simulink model "experiment_supervisor"  (R2026b)
settings: Solver=FixedStepDiscrete  StopTime=inf  FixedStep=Ts
model workspace (MAT data in the model file):
  CAN_ANGLE_DEG2ICUB = Simulink.Parameter
  CAN_ANGLE_DEG2ICUB.Value = 182.044449
  CAN_ANGLE_DEG2ICUB.Complexity = 'real'
  CAN_ANGLE_DEG2ICUB.Dimensions = [1 1]
  CAN_ANGLE_DEG2ICUB.DataType = 'single'
  CAN_ANGLE_ICUB2DEG = Simulink.Parameter
  CAN_ANGLE_ICUB2DEG.Value = 0.00549316406
  CAN_ANGLE_ICUB2DEG.Complexity = 'real'
  CAN_ANGLE_ICUB2DEG.Dimensions = [1 1]
  CAN_ANGLE_ICUB2DEG.DataType = 'single'
  Ts = Simulink.Parameter
  Ts.Value = 0.01
  Ts.Complexity = 'real'
  Ts.Dimensions = [1 1]
  Ts.DocUnits = 's'
  board_ID = Simulink.Parameter
  board_ID.Value = 1
  board_ID.Complexity = 'real'
  board_ID.Dimensions = [1 1]
undefined symbols (not defined in the file or in its folder): canChannel
libraries: canmsglib x20, canlib x4, simulink x1
settings Model: DataDictionary=amcmj1.sldd  Creator=upattacini  LastModifiedBy=ksangalli
settings SolverCC: DecoupledContinuousIntegration=on  MinimalZcImpactIntegration=on
settings OptimizationCC: ReuseModelBlockBuffer=off  SimCompilerOptimization=on
settings DebuggingCC: ArithmeticOperatorsInVariantConditions=warning  ParameterPrecisionLossMsg=none
settings HardwareCC: ProdHWDeviceType=Intel->x86-64 (Linux 64)  ProdLongLongMode=on
settings SFSimCC: CustomCodeUndefinedFunction=UseInterfaceOnly  SimUseLocalCustomCode=off
settings RTWCC: DLArmComputeVersion=19.05  Description=Simulink Desktop Real-Time  RTWCompilerOptimization=on  RTWUseLocalCustomCode=off  SystemTargetFile=sldrt.tlc  TemplateMakefile=sldrt.tmf
settings SimulinkDesktopRealTimeCC: ParMdlRefBuildCompliant=on  RealTimeExecution=kernel  TargetLibSuffix=_sldrt.a  TargetPreCompLibLocation=C:\Program Files\MATLAB\R2026b\toolbox\sldrt\lib\win64

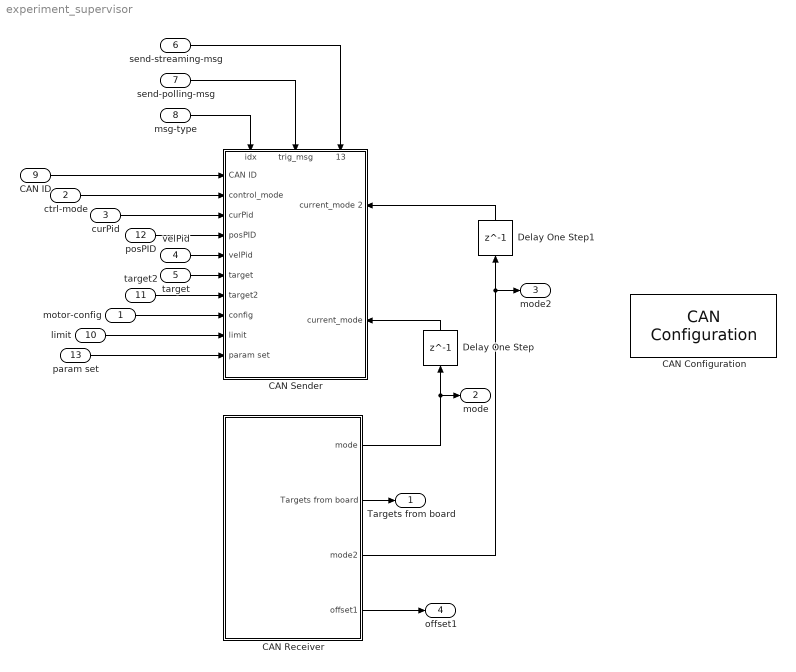
== system experiment_supervisor ==
  motor-config : Inport  OutDataTypeStr=Bus: MotorConfigurationExternal
  ctrl-mode : Inport  Port=2  OutDataTypeStr=Enum: MCControlModes
  curPid : Inport  Port=3  OutDataTypeStr=Bus: PID
  velPid : Inport  Port=4  OutDataTypeStr=Bus: PID
  target : Inport  Port=5
  send-streaming-msg : Inport  Port=6  OutDataTypeStr=uint8
  send-polling-msg : Inport  Port=7  OutDataTypeStr=uint8
  msg-type : Inport  Port=8  OutDataTypeStr=uint8
  CAN ID : Inport  Port=9
  limit : Inport  Port=10
  target2 : Inport  Port=11
  posPID : Inport  Port=12  OutDataTypeStr=Bus: PID
  param set : Inport  Port=13  OutDataTypeStr=Bus: MotorConfigurationExtSet
  CAN Configuration : canlib/CAN Configuration  BlockHandle=2987.0028  Device=Vector VN1610 1 (Channel 1)  DeviceMenu=Vector VN1610 1 (Channel 1)  ObjConstructor=canChannel('Vector', 'VN1610 1', 1)  BusSpeed=1000000  EnableBitParameters=off  SJW=1  TSEG1=4  TSEG2=3  NSamples=1  AckMode=Normal
  CAN Receiver : Subsystem
  CAN Sender : Subsystem
      settings: PortSchema="{\"entries\":[{\"content\":{\"sides\":[{\"content\":{\"connectorIds\":[\"In1\",\"In2\",\"In3\",\"In4\",\"In5\",\"In6\",\"In7\",\"In8\",\"In9\",\"In10\"]},\"type\":\"ConnectorPlacement.EquallySpacedRectSide\",\"uuid\":\"bdd6ce9e-9b65-4aba-9b48-f09f8c1326bb\"},{\"content\":{\"connectorIds\":[\"In14\",\"In15\"],\"side\":\"RIGHT\"},\"type\":\"ConnectorPlacement.EquallySpacedRectSide\",\"uuid\":\"141c9ef5-f742-47fc-b635-015c7474b58f\"},{\"content\":{\"connectorIds\":[\"In11\",\"In12\",\"In13\"],\"side\":\"TOP\"},\"type\":\"ConnectorPlacement.EquallySpacedRectSide\",\"uuid\":\"624889ac-74c5-4b05-9d21-0587daea952f\"}]},\"type\":\"ConnectorPlacement.EquallySpacedConnector\",\"uuid\":\"a748afda-e52d-41b4-a312-ee668058905d\"}],\"packageUris\":[\"http://schema.mathworks.com/mf0/Connector/R2020b\"],\"version\":\"1.0\"}"
  Delay One Step : Delay  DelayLength=1
  Delay One Step1 : Delay  DelayLength=1
  Targets from board : Outport
  mode : Outport  Port=2
  mode2 : Outport  Port=3
  offset1 : Outport  Port=4
  wires:
  ctrl-mode/1 -> CAN Sender/2(control_mode)
  send-streaming-msg/1 -> CAN Sender/13(trig_periodic)
  CAN Receiver/2(Targets from board) -> Targets from board/1
  velPid/1 -> CAN Sender/5(velPid)
  curPid/1 -> CAN Sender/3(curPid)
  motor-config/1 -> CAN Sender/8(config)
  CAN Receiver/1(mode) -> mode/1, Delay One Step/1
  Delay One Step/1 -> CAN Sender/15(current_mode)
  send-polling-msg/1 -> CAN Sender/12(trig_msg)
  msg-type/1 -> CAN Sender/11(idx)
  target/1 -> CAN Sender/6(target)
  CAN ID/1 -> CAN Sender/1(CAN ID)
  limit/1 -> CAN Sender/9(limit)
  CAN Receiver/4(offset1) -> offset1/1
  CAN Receiver/3(mode2) -> mode2/1, Delay One Step1/1
  Delay One Step1/1 -> CAN Sender/14(current_mode 2)
  target2/1 -> CAN Sender/7(target2)
  posPID/1 -> CAN Sender/4(posPID)
  param set/1 -> CAN Sender/10(param set)

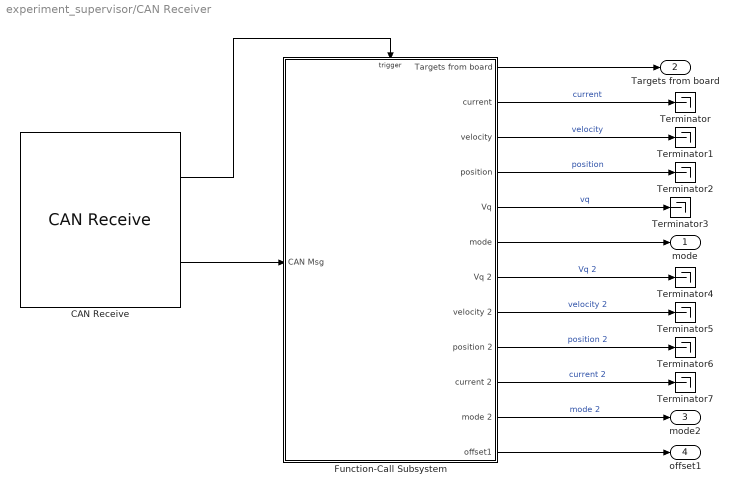
== system experiment_supervisor/CAN Receiver ==
  CAN Receive : canlib/CAN Receive  BlockHandle=2993.0018  Device=Vector VN1610 1 (Channel 1)  DeviceMenu=Vector VN1610 1 (Channel 1)  ObjConstructor=canChannel('Vector', 'VN1610 1', 1)  EnableStandardIDsFilter=off  StdIDsCombo=Allow all  StandardIDs=0  EnableExtendedIDsFilter=off  ExtIDsCombo=Allow all  ExtendedIDs=0  SampleTime=Ts  MsgsPerTimestep=all  InternalFilterUpdateStatus=on  BusOutput=on
  Function-Call Subsystem : Subsystem  TreatAsAtomicUnit=on
  Terminator{,1..7} (8 alike) : Terminator
  mode : Outport
  Targets from board : Outport  Port=2
  mode2 : Outport  Port=3
  offset1 : Outport  Port=4
  wires:
  CAN Receive/1 -> Function-Call Subsystem/Trigger
  CAN Receive/2 -> Function-Call Subsystem/1(CAN Msg)
  Function-Call Subsystem/2(current) -> Terminator/1  "current"
  Function-Call Subsystem/3(velocity) -> Terminator1/1  "velocity"
  Function-Call Subsystem/4(position) -> Terminator2/1  "position"
  Function-Call Subsystem/5(Vq) -> Terminator3/1  "vq"
  Function-Call Subsystem/1(Targets from board) -> Targets from board/1
  Function-Call Subsystem/6(mode) -> mode/1
  Function-Call Subsystem/7(Vq 2) -> Terminator4/1  "Vq 2"
  Function-Call Subsystem/8(velocity 2) -> Terminator5/1  "velocity 2"
  Function-Call Subsystem/9(position 2) -> Terminator6/1  "position 2"
  Function-Call Subsystem/10(current 2) -> Terminator7/1  "current 2"
  Function-Call Subsystem/11(mode 2) -> mode2/1  "mode 2"
  Function-Call Subsystem/12(offset1) -> offset1/1

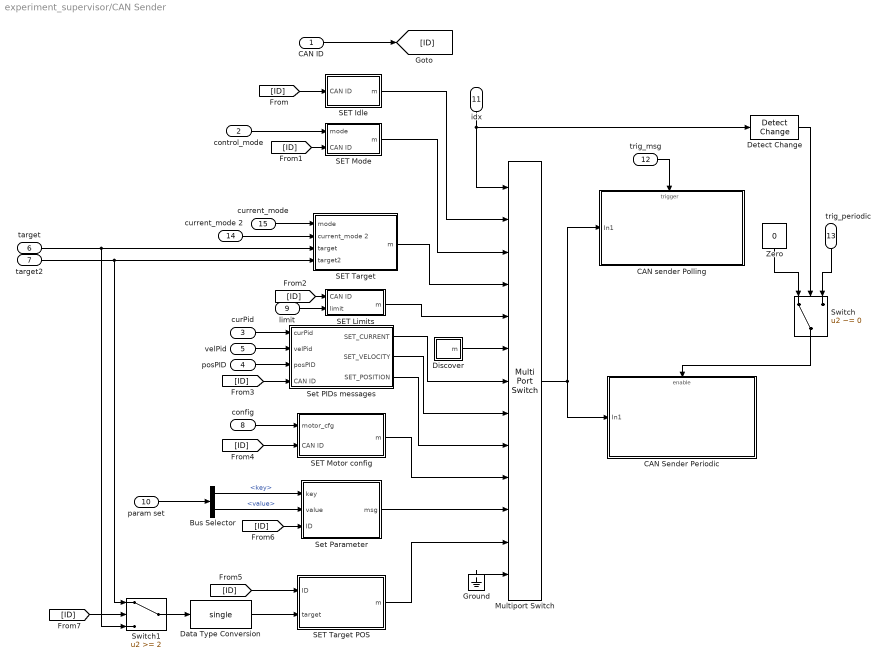
== system experiment_supervisor/CAN Sender ==
  CAN ID : Inport
  control_mode : Inport  Port=2
  curPid : Inport  Port=3
  posPID : Inport  Port=4
  velPid : Inport  Port=5
  target : Inport  Port=6
  target2 : Inport  Port=7
  config : Inport  Port=8
  limit : Inport  Port=9
  param set : Inport  Port=10  OutDataTypeStr=Bus: MotorConfigurationExtSet
  idx : Inport  Port=11
  trig_msg : Inport  Port=12
  trig_periodic : Inport  Port=13
  current_mode 2 : Inport  Port=14
  current_mode : Inport  Port=15
  Bus Selector : BusSelector  OutputSignals=key,value
  CAN Sender Periodic : Subsystem  TreatAsAtomicUnit=on
  CAN sender Polling : Subsystem
  Data Type Conversion : DataTypeConversion  OutDataTypeStr=single  SaturateOnIntegerOverflow=off  RndMeth=Floor
  Detect Change : simulink/Logic and Bit Operations/Detect Change  vinit=0  OutDataTypeStr=boolean
  Discover : Subsystem
  Ground : Ground
  Multiport Switch : MultiPortSwitch  Inputs=12  DiagnosticForDefault=Warning  SaturateOnIntegerOverflow=off  InputSameDT=off
  SET Idle : Subsystem
  SET Limits : Subsystem
  SET Mode : Subsystem
  SET Motor config : Subsystem
  SET Target : Subsystem
  "SET Target POS " : Subsystem
  Set PIDs messages : Subsystem
  Set Parameter : Subsystem
  Switch : Switch  Criteria=u2 ~= 0  SaturateOnIntegerOverflow=off  InputSameDT=off
  Switch1 : Switch  Threshold=2  SaturateOnIntegerOverflow=off  InputSameDT=off
  Zero : Constant  Value=0  OutDataTypeStr=Inherit: Inherit via back propagation
  wires:
  idx/1 -> Multiport Switch/1, Detect Change/1
  trig_msg/1 -> CAN sender Polling/Trigger
  trig_periodic/1 -> Switch/3
  Multiport Switch/1 -> CAN sender Polling/1(In1), CAN Sender Periodic/1(In1)
  Set PIDs messages/2(SET_VELOCITY) -> Multiport Switch/8
  Set PIDs messages/1(SET_CURRENT) -> Multiport Switch/7
  velPid/1 -> Set PIDs messages/2(velPid)
  curPid/1 -> Set PIDs messages/1(curPid)
  Detect Change/1 -> Switch/2
  Zero/1 -> Switch/1
  Switch/1 -> CAN Sender Periodic/Enable
  SET Limits/1(m) -> Multiport Switch/5
  current_mode/1 -> SET Target/1(mode)
  target/1 -> Switch1/3, SET Target/3(target)
  SET Target/1(m) -> Multiport Switch/4
  config/1 -> SET Motor config/1(motor_cfg)
  control_mode/1 -> SET Mode/1(mode)
  SET Mode/1(m) -> Multiport Switch/3
  SET Idle/1(m) -> Multiport Switch/2
  Discover/1(m) -> Multiport Switch/6
  [ID] -> SET Idle/1(CAN ID)
  [ID] -> SET Mode/2(CAN ID)
  [ID] -> SET Limits/1(CAN ID)
  [ID] -> Set PIDs messages/4(CAN ID)
  [ID] -> SET Motor config/2(CAN ID)
  CAN ID/1 -> [ID]
  limit/1 -> SET Limits/2(limit)
  current_mode 2/1 -> SET Target/2(current_mode 2)
  target2/1 -> Switch1/1, SET Target/4(target2)
  posPID/1 -> Set PIDs messages/3(posPID)
  [ID] -> "SET Target POS "/1(ID)
  "SET Target POS "/1(m) -> Multiport Switch/12
  Data Type Conversion/1 -> "SET Target POS "/2(target)
  Set PIDs messages/3(SET_POSITION) -> Multiport Switch/9
  SET Motor config/1(m) -> Multiport Switch/10
  param set/1 -> Bus Selector/1
  Ground/1 -> Multiport Switch/13
  Bus Selector/1 -> Set Parameter/1(key)  "<key>"
  Bus Selector/2 -> Set Parameter/2(value)  "<value>"
  [ID] -> Set Parameter/3(ID)
  Set Parameter/1(msg) -> Multiport Switch/11
  Switch1/1 -> Data Type Conversion/1
  [ID] -> Switch1/2

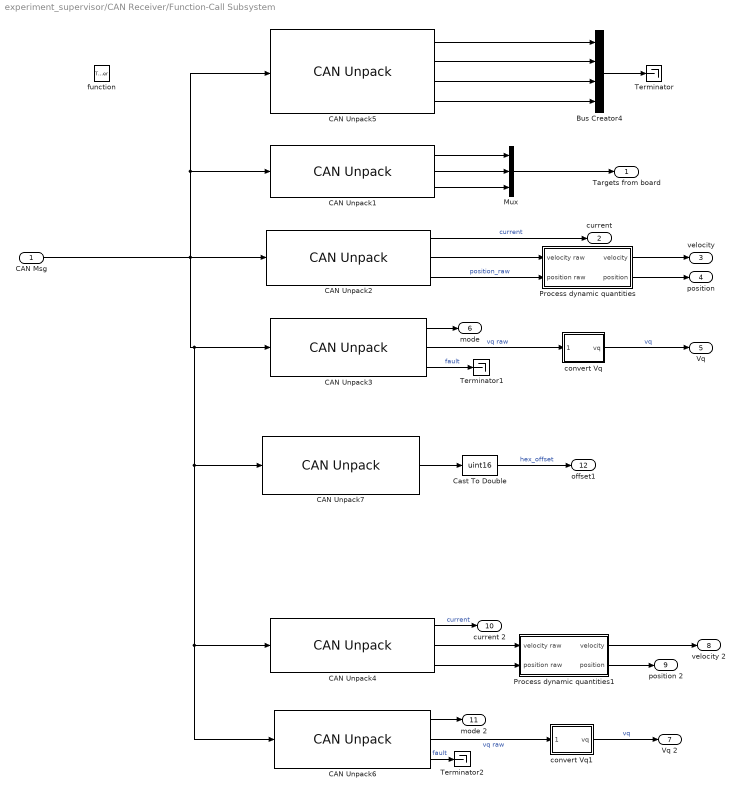
== system experiment_supervisor/CAN Receiver/Function-Call Subsystem ==
  CAN Msg : Inport
  function : TriggerPort  TriggerType=function-call  VariantControl=(inherit)
  Bus Creator4 : BusCreator  Inputs=4
  CAN Unpack1 : canmsglib/CAN Unpack  MsgList=(none)  MsgName=TARGETS  MsgIDType=Standard (11-bit identifier)  MsgIdentifier=0x10F  MsgLength=8  SignalInfo={ 'Target1', '0', '16', 'LE', 'signed', 'Standard', '0', '1', '0', '-Inf', 'Inf'; 'Target2', '16', '16', 'LE', 'signed', 'Standard', '0', '1', '0', '-Inf', 'Inf'; 'Target3', '32', '16', 'LE', 'signed', 'Standard', '0', '1', '0', '-Inf', 'Inf' }  IDPort=off  TimestampPort=off  ErrorPort=off  RemotePort=off  LengthPort=off  StatusPort=off  ApplyMinMax=off
  CAN Unpack2 : canmsglib/CAN Unpack  MsgList=(none)  MsgName=FOC  MsgIDType=Standard (11-bit identifier)  MsgIdentifier=0x110  MsgLength=8  SignalInfo={ 'current', '0', '16', 'LE', 'signed', 'Standard', '0', '1', '0', '-Inf', 'Inf'; 'velocity', '16', '16', 'LE', 'signed', 'Standard', '0', '1', '0', '-Inf', 'Inf'; 'position', '32', '32', 'LE', 'signed', 'Standard', '0', '1', '0', '-Inf', 'Inf' }  IDPort=off  TimestampPort=off  ErrorPort=off  RemotePort=off  LengthPort=off  StatusPort=off  ApplyMinMax=off
  CAN Unpack3 : canmsglib/CAN Unpack  MsgList=(none)  MsgName=STATUS  MsgIDType=Standard (11-bit identifier)  MsgIdentifier=0x113  MsgLength=8  SignalInfo={ 'mode', '0', '8', 'LE', 'unsigned', 'Standard', '0', '1', '0', '-Inf', 'Inf'; 'pwm', '16', '16', 'LE', 'unsigned', 'Standard', '0', '1', '0', '-Inf', 'Inf'; 'fault', '32', '8', 'LE', 'unsigned', 'Standard', '0', '1', '0', '-Inf', 'Inf' }  IDPort=off  TimestampPort=off  ErrorPort=off  RemotePort=off  LengthPort=off  StatusPort=off  ApplyMinMax=off
  CAN Unpack4 : canmsglib/CAN Unpack  MsgList=(none)  MsgName=FOC  MsgIDType=Standard (11-bit identifier)  MsgIdentifier=0x120  MsgLength=8  SignalInfo={ 'current', '0', '16', 'LE', 'signed', 'Standard', '0', '1', '0', '-Inf', 'Inf'; 'velocity', '16', '16', 'LE', 'signed', 'Standard', '0', '1', '0', '-Inf', 'Inf'; 'position', '32', '32', 'LE', 'signed', 'Standard', '0', '1', '0', '-Inf', 'Inf' }  IDPort=off  TimestampPort=off  ErrorPort=off  RemotePort=off  LengthPort=off  StatusPort=off  ApplyMinMax=off
  CAN Unpack5 : canmsglib/CAN Unpack  MsgList=(none)  MsgName=DISCOVER  MsgIDType=Standard (11-bit identifier)  MsgIdentifier=0x710  MsgLength=5  SignalInfo={}  IDPort=on  TimestampPort=on  ErrorPort=off  RemotePort=off  LengthPort=on  StatusPort=off  ApplyMinMax=off
      settings: DataFormat=raw data
  CAN Unpack6 : canmsglib/CAN Unpack  MsgList=(none)  MsgName=STATUS  MsgIDType=Standard (11-bit identifier)  MsgIdentifier=0x123  MsgLength=8  SignalInfo={ 'mode', '0', '8', 'LE', 'unsigned', 'Standard', '0', '1', '0', '-Inf', 'Inf'; 'pwm', '16', '16', 'LE', 'unsigned', 'Standard', '0', '1', '0', '-Inf', 'Inf'; 'fault', '32', '8', 'LE', 'unsigned', 'Standard', '0', '1', '0', '-Inf', 'Inf' }  IDPort=off  TimestampPort=off  ErrorPort=off  RemotePort=off  LengthPort=off  StatusPort=off  ApplyMinMax=off
  CAN Unpack7 : canmsglib/CAN Unpack  MsgList=(none)  MsgName=Debug  MsgIDType=Standard (11-bit identifier)  MsgIdentifier=0x119  MsgLength=8  SignalInfo={ 'offset', '0', '16', 'LE', 'unsigned', 'Standard', '0', '1', '0', '-Inf', 'Inf' }  IDPort=off  TimestampPort=off  ErrorPort=off  RemotePort=off  LengthPort=off  StatusPort=off  ApplyMinMax=off
  Cast To Double : DataTypeConversion  OutDataTypeStr=uint16  SaturateOnIntegerOverflow=off  RndMeth=Floor
  Mux : Mux  Inputs=3
  Process dynamic quantities : Subsystem
  Process dynamic quantities1 : Subsystem
  Terminator : Terminator
  Terminator1 : Terminator
  Terminator2 : Terminator
  convert Vq : Subsystem
  convert Vq1 : Subsystem
  Targets from board : Outport
  current : Outport  Port=2  Unit=mA
  velocity : Outport  Port=3  Unit=deg/s
  position : Outport  Port=4  Unit=deg
  Vq : Outport  Port=5  Unit=%  PortDimensions=1
  mode : Outport  Port=6  OutDataTypeStr=uint8
  Vq 2 : Outport  Port=7
  velocity 2 : Outport  Port=8
  position 2 : Outport  Port=9
  current 2 : Outport  Port=10  Unit=mA
  mode 2 : Outport  Port=11  OutDataTypeStr=uint8
  offset1 : Outport  Port=12
  wires:
  CAN Unpack5/4 -> Bus Creator4/4
  CAN Unpack5/3 -> Bus Creator4/3
  CAN Unpack5/2 -> Bus Creator4/2
  CAN Unpack5/1 -> Bus Creator4/1
  Bus Creator4/1 -> Terminator/1
  CAN Unpack1/1 -> Mux/1
  CAN Unpack1/2 -> Mux/2
  CAN Unpack1/3 -> Mux/3
  Mux/1 -> Targets from board/1
  CAN Unpack2/2 -> Process dynamic quantities/1(velocity raw)
  Process dynamic quantities/2(position) -> position/1
  Process dynamic quantities/1(velocity) -> velocity/1
  CAN Unpack2/3 -> Process dynamic quantities/2(position raw)  "position_raw"
  CAN Unpack3/2 -> convert Vq/1(vq raw)  "vq raw"
  CAN Unpack3/1 -> mode/1
  convert Vq/1(vq) -> Vq/1  "vq"
  CAN Unpack3/3 -> Terminator1/1  "fault"
  CAN Msg/1 -> CAN Unpack5/1, CAN Unpack1/1, CAN Unpack7/1, CAN Unpack6/1, CAN Unpack4/1, CAN Unpack3/1, CAN Unpack2/1
  CAN Unpack4/2 -> Process dynamic quantities1/1(velocity raw)
  CAN Unpack4/3 -> Process dynamic quantities1/2(position raw)
  CAN Unpack6/2 -> convert Vq1/1(vq raw)  "vq raw"
  Process dynamic quantities1/1(velocity) -> velocity 2/1
  Process dynamic quantities1/2(position) -> position 2/1
  convert Vq1/1(vq) -> Vq 2/1  "vq"
  CAN Unpack4/1 -> current 2/1  "current"
  CAN Unpack6/1 -> mode 2/1
  CAN Unpack6/3 -> Terminator2/1  "fault"
  CAN Unpack7/1 -> Cast To Double/1
  Cast To Double/1 -> offset1/1  "hex_offset"
  CAN Unpack2/1 -> current/1  "current"

== system experiment_supervisor/CAN Sender/CAN Sender Periodic ==
  In1 : Inport
  Enable : EnablePort
  CAN Transmit : canlib/CAN Transmit  BlockHandle=1809.0078  Device=Vector VN1610 1 (Channel 1)  DeviceMenu=Vector VN1610 1 (Channel 1)  ObjConstructor=canChannel('Vector', 'VN1610 1', 1)  EnableEventTransmit=off  EnablePeriodicTransmit=on  MessagePeriod=Ts
  wires:
  In1/1 -> CAN Transmit/1

== system experiment_supervisor/CAN Sender/CAN sender Polling ==
  In1 : Inport
  Trigger : TriggerPort  VariantControl=(inherit)  PortDimensions=1
  CAN Transmit : canlib/CAN Transmit  BlockHandle=1818.0078  Device=Vector VN1610 1 (Channel 1)  DeviceMenu=Vector VN1610 1 (Channel 1)  ObjConstructor=canChannel('Vector', 'VN1610 1', 1)  EnableEventTransmit=off  EnablePeriodicTransmit=off  MessagePeriod=1.000
  wires:
  In1/1 -> CAN Transmit/1

== system experiment_supervisor/CAN Sender/Discover ==
  CAN Pack4 : canmsglib/CAN Pack  MsgList=(none)  MsgName=DISCOVER  MsgIDType=Standard (11-bit identifier)  MsgIdentifier=0x70F  CANIDInput=off  MsgLength=1  Remote=off  ApplyMinMax=off  BusOutput=on  SignalInfo={}
      settings: DataFormat=raw data
  discover : Constant  Value=0xFF
  m : Outport
  wires:
  CAN Pack4/1 -> m/1
  discover/1 -> CAN Pack4/1

== system experiment_supervisor/CAN Sender/SET Idle ==
  CAN ID : Inport
  CAN Pack : canmsglib/CAN Pack  MsgList=(none)  MsgName=CAN Idle  MsgIDType=Standard (11-bit identifier)  MsgIdentifier=board_ID  CANIDInput=on  MsgLength=2  Remote=off  ApplyMinMax=off  BusOutput=on  SignalInfo={ 'Idle', '0', '16', 'LE', 'unsigned', 'Standard', '0', '1', '0', '-Inf', 'Inf' }
      settings: DataFormat=manually specified signals
  idle-mode : Constant  Value=0x09  OutDataTypeStr=Inherit: Inherit via back propagation
  m : Outport
  wires:
  idle-mode/1 -> CAN Pack/1
  CAN ID/1 -> CAN Pack/2
  CAN Pack/1 -> m/1

== system experiment_supervisor/CAN Sender/SET Limits ==
  CAN ID : Inport
  limit : Inport  Port=2
  CAN Pack3 : canmsglib/CAN Pack  MsgList=(none)  MsgName=CAN Limits  MsgIDType=Standard (11-bit identifier)  MsgIdentifier=board_ID  CANIDInput=on  MsgLength=8  Remote=off  ApplyMinMax=off  BusOutput=on  SignalInfo={ 'CMD', '0', '8', 'LE', 'unsigned', 'Standard', '0', '1', '0', '-Inf', 'Inf'; 'X', '8', '8', 'LE', 'unsigned', 'Standard', '0', '1', '0', '-Inf', 'Inf'; 'NOMINAL', '16', '16', 'LE', 'unsigned', 'Standard', '0', '1', '0', '-Inf', 'Inf'; 'PEAK', '32', '16', 'LE', 'unsigned', 'Standard', '0', '1', '0', '-Inf', 'Inf'; 'OVERLOAD', '48', '16', 'LE', 'unsigned', 'Standard', '0', '1', '0', '-Inf', 'Inf' }
      settings: DataFormat=manually specified signals
  Constant1 : Constant  Value=0x48  OutDataTypeStr=Inherit: Inherit via back propagation
  Constant2 : Constant  Value=0  OutDataTypeStr=Inherit: Inherit via back propagation
  Demux : Demux  Outputs=3
  m : Outport
  wires:
  Constant2/1 -> CAN Pack3/2
  Constant1/1 -> CAN Pack3/1
  Demux/1 -> CAN Pack3/3
  Demux/3 -> CAN Pack3/5
  Demux/2 -> CAN Pack3/4
  CAN ID/1 -> CAN Pack3/6
  CAN Pack3/1 -> m/1
  limit/1 -> Demux/1

== system experiment_supervisor/CAN Sender/SET Mode ==
  mode : Inport
  CAN ID : Inport  Port=2
  CAN Pack1 : canmsglib/CAN Pack  MsgList=(none)  MsgName=SET Control Mode  MsgIDType=Standard (11-bit identifier)  MsgIdentifier=board_ID  CANIDInput=on  MsgLength=2  Remote=off  ApplyMinMax=off  BusOutput=on  SignalInfo={ 'CMD', '0', '8', 'LE', 'unsigned', 'Standard', '0', '1', '0', '-Inf', 'Inf'; 'CTRL', '8', '8', 'LE', 'signed', 'Standard', '0', '1', '0', '-Inf', 'Inf' }
      settings: DataFormat=manually specified signals
  Cast : DataTypeConversion  OutDataTypeStr=uint8  SaturateOnIntegerOverflow=off  RndMeth=Floor
  current-mode : Constant  Value=0x09  OutDataTypeStr=Inherit: Inherit via back propagation
  m : Outport
  wires:
  current-mode/1 -> CAN Pack1/1
  Cast/1 -> CAN Pack1/2
  mode/1 -> Cast/1
  CAN ID/1 -> CAN Pack1/3
  CAN Pack1/1 -> m/1

== system experiment_supervisor/CAN Sender/SET Motor config ==
  motor_cfg : Inport
  CAN ID : Inport  Port=2
  CAN Pack5 : canmsglib/CAN Pack  MsgList=(none)  MsgName=Set_Motor_Config  MsgIDType=Standard (11-bit identifier)  MsgIdentifier=board_ID  CANIDInput=on  MsgLength=8  Remote=off  ApplyMinMax=off  BusOutput=on  SignalInfo={ 'CMD', '0', '8', 'LE', 'unsigned', 'Standard', '0', '1', '0', '-Inf', 'Inf'; 'FLAGS', '8', '8', 'LE', 'unsigned', 'Standard', '0', '1', '0', '-Inf', 'Inf'; 'RES_ENCODER', '16', '16', 'LE', 'signed', 'Standard', '0', '1', '0', '-Inf', 'Inf'; 'OFFSET_ENCODER', '32', '16', 'LE', 'signed', 'Standard', '0', '1', '0', '-Inf', 'Inf'; 'N_POLES', '48', '8', 'LE', 'unsigned', 'Standard', '0', '1', '0', '-Inf', 'Inf'; 'ENCODER_TOLERANCE', '56', '8', 'LE', 'unsigned', 'Standard', '0', '1', '0', '-Inf', 'Inf' }
      settings: DataFormat=manually specified signals
  Constant3 : Constant  Value=0x77  OutDataTypeStr=Inherit: Inherit via back propagation
  Unpack motor configuration : MATLAB Function  TreatAsAtomicUnit=on
  m : Outport
  wires:
  motor_cfg/1 -> Unpack motor configuration/1(motor_cfg)
  Unpack motor configuration/2(resolution) -> CAN Pack5/3
  Unpack motor configuration/3(rotor_offset) -> CAN Pack5/4
  Unpack motor configuration/1(flags) -> CAN Pack5/2
  Unpack motor configuration/4(n_poles) -> CAN Pack5/5
  Unpack motor configuration/5(enc_tolerance) -> CAN Pack5/6
  Constant3/1 -> CAN Pack5/1
  CAN ID/1 -> CAN Pack5/7
  CAN Pack5/1 -> m/1

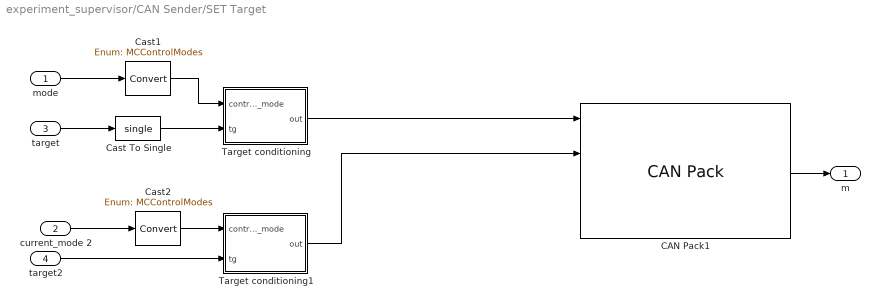
== system experiment_supervisor/CAN Sender/SET Target ==
  mode : Inport
  current_mode 2 : Inport  Port=2
  target : Inport  Port=3
  target2 : Inport  Port=4
  CAN Pack1 : canmsglib/CAN Pack  MsgList=(none)  MsgName=CAN Target  MsgIDType=Standard (11-bit identifier)  MsgIdentifier=0x10F  CANIDInput=off  MsgLength=8  Remote=off  ApplyMinMax=off  BusOutput=on  SignalInfo={ 'Target 1', '0', '16', 'LE', 'signed', 'Standard', '0', '1', '0', '-Inf', 'Inf'; 'Target 2', '16', '16', 'LE', 'signed', 'Standard', '0', '1', '0', '-Inf', 'Inf'; 'Target 3', '32', '16', 'LE', 'signed', 'Standard', '0', '1', '0', '-Inf', 'Inf'; 'Target 4', '48', '16', 'LE', 'signed', 'Standard', '0', '1', '0', '-Inf', 'Inf' }
      settings: DataFormat=manually specified signals
  Cast To Single : DataTypeConversion  OutDataTypeStr=single  SaturateOnIntegerOverflow=off  RndMeth=Floor
  Cast1 : DataTypeConversion  OutDataTypeStr=Enum: MCControlModes  SaturateOnIntegerOverflow=off  RndMeth=Floor
  Cast2 : DataTypeConversion  OutDataTypeStr=Enum: MCControlModes  SaturateOnIntegerOverflow=off  RndMeth=Floor
  Target conditioning : Subsystem
  Target conditioning1 : Subsystem
  m : Outport
  wires:
  Cast To Single/1 -> Target conditioning/2(tg)
  Cast1/1 -> Target conditioning/1(control_mode)
  target/1 -> Cast To Single/1
  mode/1 -> Cast1/1
  Target conditioning/1(out) -> CAN Pack1/1
  current_mode 2/1 -> Cast2/1
  target2/1 -> Target conditioning1/2(tg)
  Cast2/1 -> Target conditioning1/1(control_mode)
  CAN Pack1/1 -> m/1
  Target conditioning1/1(out) -> CAN Pack1/2

== system experiment_supervisor/CAN Sender/SET Target POS  ==
  note: +90 0x55A0
      | 180 0x59A0
      | 2.5 0x4100
      | 6000 (1000 rpm) 0x6ddc
  ID : Inport
  target : Inport  Port=2
  CAN Pack3 : canmsglib/CAN Pack  MsgList=(none)  MsgName=SET  MsgIDType=Standard (11-bit identifier)  MsgIdentifier=board_ID  CANIDInput=on  MsgLength=8  Remote=off  ApplyMinMax=off  BusOutput=on  SignalInfo={ 'CMD', '0', '8', 'LE', 'unsigned', 'Standard', '0', '1', '0', '-Inf', 'Inf'; 'SetPos', '8', '8', 'LE', 'unsigned', 'Standard', '0', '1', '0', '-Inf', 'Inf'; 'TargetPos', '16', '32', 'LE', 'single', 'Standard', '0', '1', '0', '-Inf', 'Inf'; 'Vel', '48', '16', 'LE', 'unsigned', 'Standard', '0', '1', '0', '-Inf', 'Inf' }
      settings: DataFormat=manually specified signals
  Constant : Constant  Value=0x05
  Constant1 : Constant  Value=0x6ddc  OutDataTypeStr=uint16
  MATLAB Function : MATLAB Function  Commented=through  TreatAsAtomicUnit=on
  Target conditioning : Subsystem
  m : Outport
  wires:
  target/1 -> Target conditioning/1(tg)
  Constant/1 -> CAN Pack3/1
  CAN Pack3/1 -> m/1
  ID/1 -> CAN Pack3/5
  Target conditioning/1(ID) -> CAN Pack3/2
  Target conditioning/2(Position) -> CAN Pack3/3
  Constant1/1 -> MATLAB Function/1(u)
  MATLAB Function/1(y) -> CAN Pack3/4

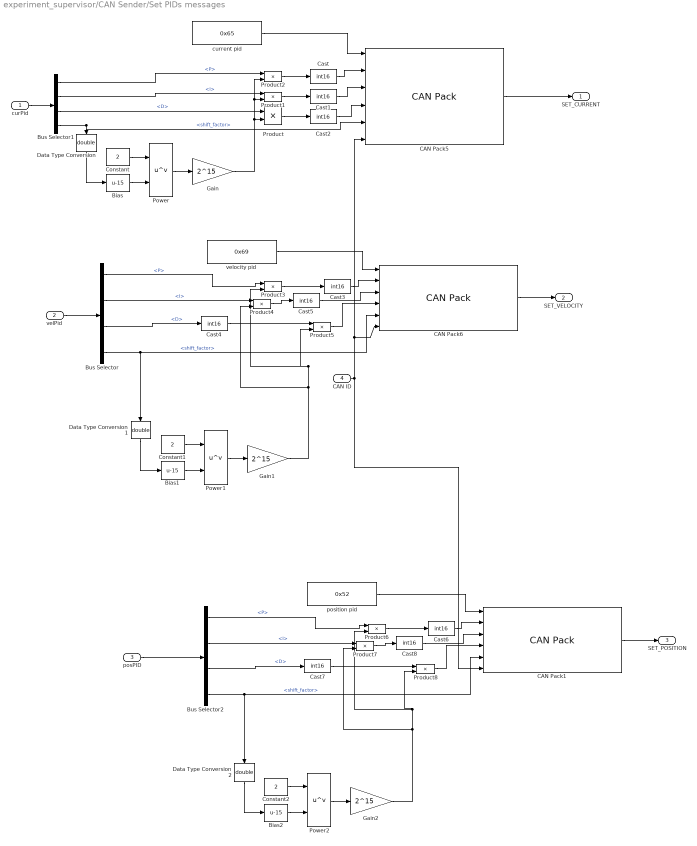
== system experiment_supervisor/CAN Sender/Set PIDs messages ==
  curPid : Inport
  velPid : Inport  Port=2
  posPID : Inport  Port=3
  CAN ID : Inport  Port=4
  Bias : Bias  Bias=-15  SaturateOnIntegerOverflow=off
  Bias1 : Bias  Bias=-15  SaturateOnIntegerOverflow=off
  Bias2 : Bias  Bias=-15  SaturateOnIntegerOverflow=off
  Bus Selector : BusSelector  OutputSignals=P,I,D,shift_factor
  Bus Selector1 : BusSelector  OutputSignals=P,I,D,shift_factor
  Bus Selector2 : BusSelector  OutputSignals=P,I,D,shift_factor
  CAN Pack1 : canmsglib/CAN Pack  MsgList=(none)  MsgName=SET_POSITION_PID  MsgIDType=Standard (11-bit identifier)  MsgIdentifier=board_ID  CANIDInput=on  MsgLength=8  Remote=off  ApplyMinMax=off  BusOutput=on  SignalInfo={ 'CMD', '0', '8', 'LE', 'unsigned', 'Standard', '0', '1', '0', '-Inf', 'Inf'; 'Kp', '8', '16', 'LE', 'signed', 'Standard', '0', '1', '0', '-Inf', 'Inf'; 'Ki', '24', '16', 'LE', 'signed', 'Standard', '0', '1', '0', '-Inf', 'Inf'; 'Kd', '40', '16', 'LE', 'signed', 'Standard', '0', '1', '0', '-Inf', 'Inf'; 'shift', '56', '8', 'LE', 'unsigned', 'Standard', '0', '1', '0', '-Inf', 'Inf' }
      settings: DataFormat=manually specified signals
  CAN Pack5 : canmsglib/CAN Pack  MsgList=(none)  MsgName=SET_CURRENT_PID  MsgIDType=Standard (11-bit identifier)  MsgIdentifier=board_ID  CANIDInput=on  MsgLength=8  Remote=off  ApplyMinMax=off  BusOutput=on  SignalInfo={ 'CMD', '0', '8', 'LE', 'unsigned', 'Standard', '0', '1', '0', '-Inf', 'Inf'; 'Kp', '8', '16', 'LE', 'signed', 'Standard', '0', '1', '0', '-Inf', 'Inf'; 'Ki', '24', '16', 'LE', 'signed', 'Standard', '0', '1', '0', '-Inf', 'Inf'; 'Kd', '40', '16', 'LE', 'signed', 'Standard', '0', '1', '0', '-Inf', 'Inf'; 'shift', '56', '8', 'LE', 'unsigned', 'Standard', '0', '1', '0', '-Inf', 'Inf' }
      settings: DataFormat=manually specified signals
  CAN Pack6 : canmsglib/CAN Pack  MsgList=(none)  MsgName=SET_VELOCITY_PID  MsgIDType=Standard (11-bit identifier)  MsgIdentifier=board_ID  CANIDInput=on  MsgLength=8  Remote=off  ApplyMinMax=off  BusOutput=on  SignalInfo={ 'CMD', '0', '8', 'LE', 'unsigned', 'Standard', '0', '1', '0', '-Inf', 'Inf'; 'Kp', '8', '16', 'LE', 'signed', 'Standard', '0', '1', '0', '-Inf', 'Inf'; 'Ki', '24', '16', 'LE', 'signed', 'Standard', '0', '1', '0', '-Inf', 'Inf'; 'Kd', '40', '16', 'LE', 'signed', 'Standard', '0', '1', '0', '-Inf', 'Inf'; 'shift', '56', '8', 'LE', 'unsigned', 'Standard', '0', '1', '0', '-Inf', 'Inf' }
      settings: DataFormat=manually specified signals
  Cast{,1..8} (9 alike) : DataTypeConversion  OutDataTypeStr=int16  SaturateOnIntegerOverflow=off  RndMeth=Floor
  Constant : Constant  Value=2
  Constant1 : Constant  Value=2
  Constant2 : Constant  Value=2
  Data Type Conversion : DataTypeConversion  OutDataTypeStr=double  SaturateOnIntegerOverflow=off  RndMeth=Floor
  Data Type Conversion1 : DataTypeConversion  OutDataTypeStr=double  SaturateOnIntegerOverflow=off  RndMeth=Floor
  Data Type Conversion2 : DataTypeConversion  OutDataTypeStr=double  SaturateOnIntegerOverflow=off  RndMeth=Floor
  Gain : Gain  Gain=2^15  OutDataTypeStr=single
  Gain1 : Gain  Gain=2^15  OutDataTypeStr=single
  Gain2 : Gain  Gain=2^15  OutDataTypeStr=single
  Power : Math  Operator=pow
  Power1 : Math  Operator=pow
  Power2 : Math  Operator=pow
  Product{,1..8} (9 alike) : Product
  current pid : Constant  Value=0x65  OutDataTypeStr=int16
  position pid : Constant  Value=0x52  OutDataTypeStr=int16
  velocity pid : Constant  Value=0x69  OutDataTypeStr=int16
  SET_CURRENT : Outport
  SET_VELOCITY : Outport  Port=2
  SET_POSITION : Outport  Port=3
  wires:
  Bus Selector/4 -> CAN Pack6/5, Data Type Conversion1/1  "<shift_factor>"
  Bus Selector1/4 -> CAN Pack5/5, Data Type Conversion/1  "<shift_factor>"
  Bus Selector1/1 -> Product2/1  "<P>"
  Bus Selector1/2 -> Product1/1  "<I>"
  current pid/1 -> CAN Pack5/1
  velocity pid/1 -> CAN Pack6/1
  CAN Pack5/1 -> SET_CURRENT/1
  CAN Pack6/1 -> SET_VELOCITY/1
  velPid/1 -> Bus Selector/1
  curPid/1 -> Bus Selector1/1
  Bus Selector1/3 -> Product/1  "<D>"
  Power/1 -> Gain/1
  Gain/1 -> Product2/2, Product1/2, Product/2
  Product/1 -> Cast2/1
  Product1/1 -> Cast1/1
  Product2/1 -> Cast/1
  Cast/1 -> CAN Pack5/2
  Cast1/1 -> CAN Pack5/3
  Cast2/1 -> CAN Pack5/4
  Constant/1 -> Power/1
  Bias/1 -> Power/2
  Data Type Conversion/1 -> Bias/1
  Cast5/1 -> CAN Pack6/3
  Bus Selector/2 -> Product4/1  "<I>"
  Cast3/1 -> CAN Pack6/2
  Bus Selector/3 -> Cast4/1  "<D>"
  Bus Selector/1 -> Product3/1  "<P>"
  Cast4/1 -> Product5/1
  CAN ID/1 -> CAN Pack6/6, CAN Pack5/6, CAN Pack1/6
  Power1/1 -> Gain1/1
  Data Type Conversion1/1 -> Bias1/1
  Gain1/1 -> Product5/2, Product3/2, Product4/2
  Constant1/1 -> Power1/1
  Bias1/1 -> Power1/2
  Product3/1 -> Cast3/1
  Product4/1 -> Cast5/1
  Product5/1 -> CAN Pack6/4
  Data Type Conversion2/1 -> Bias2/1
  Gain2/1 -> Product8/2, Product6/2, Product7/2
  Bias2/1 -> Power2/2
  Power2/1 -> Gain2/1
  Product6/1 -> Cast6/1
  Cast6/1 -> CAN Pack1/2
  Cast8/1 -> CAN Pack1/3
  Constant2/1 -> Power2/1
  Bus Selector2/3 -> Cast7/1  "<D>"
  Bus Selector2/2 -> Product7/1  "<I>"
  Bus Selector2/4 -> CAN Pack1/5, Data Type Conversion2/1  "<shift_factor>"
  Bus Selector2/1 -> Product6/1  "<P>"
  position pid/1 -> CAN Pack1/1
  Product8/1 -> CAN Pack1/4
  CAN Pack1/1 -> SET_POSITION/1
  Cast7/1 -> Product8/1
  Product7/1 -> Cast8/1
  posPID/1 -> Bus Selector2/1

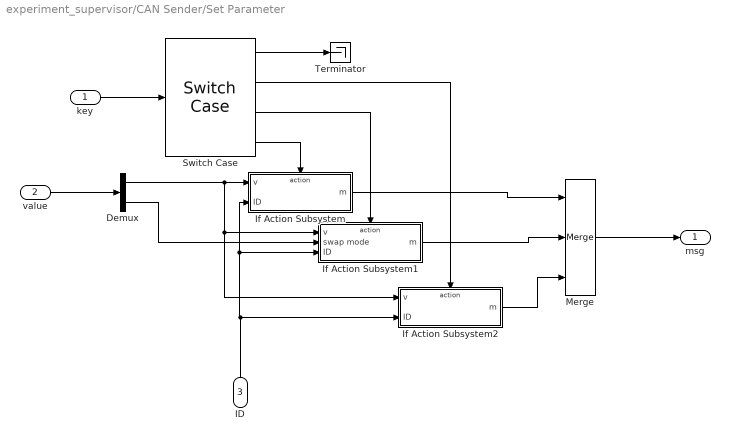
== system experiment_supervisor/CAN Sender/Set Parameter ==
  key : Inport
  value : Inport  Port=2
  ID : Inport  Port=3
  Demux : Demux  Outputs=2
  If Action Subsystem : Subsystem  TreatAsAtomicUnit=on
  If Action Subsystem1 : Subsystem  TreatAsAtomicUnit=on
  If Action Subsystem2 : Subsystem  TreatAsAtomicUnit=on
  Merge : Merge  Inputs=3
  Switch Case : SwitchCase  CaseConditions="{MCMotorParamsSet.None, MCMotorParamsSet.Kbemf, MCMotorParamsSet.hall,  MCMotorParamsSet.elect_vmax}"  ShowDefaultCase=off
  Terminator : Terminator
  msg : Outport
  wires:
  Merge/1 -> msg/1
  If Action Subsystem/1(m) -> Merge/1
  Demux/1 -> If Action Subsystem2/1(v), If Action Subsystem1/1(v), If Action Subsystem/1(v)
  key/1 -> Switch Case/1
  If Action Subsystem1/1(m) -> Merge/2
  If Action Subsystem2/1(m) -> Merge/3
  ID/1 -> If Action Subsystem/2(ID), If Action Subsystem1/3(ID), If Action Subsystem2/2(ID)
  Demux/2 -> If Action Subsystem1/2(swap mode)
  value/1 -> Demux/1
  Switch Case/2 -> If Action Subsystem2/Action
  Switch Case/3 -> If Action Subsystem1/Action
  Switch Case/4 -> If Action Subsystem/Action
  Switch Case/1 -> Terminator/1

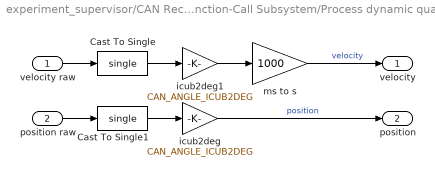
== system experiment_supervisor/CAN Receiver/Function-Call Subsystem/Process dynamic quantities ==
  velocity raw : Inport
  position raw : Inport  Port=2
  Cast To Single : DataTypeConversion  OutDataTypeStr=single  SaturateOnIntegerOverflow=off  RndMeth=Floor
  Cast To Single1 : DataTypeConversion  OutDataTypeStr=single  SaturateOnIntegerOverflow=off  RndMeth=Floor
  icub2deg : Gain  Gain=CAN_ANGLE_ICUB2DEG
  icub2deg1 : Gain  Gain=CAN_ANGLE_ICUB2DEG
  ms to s : Gain  Gain=1000
  velocity : Outport
  position : Outport  Port=2
  wires:
  Cast To Single1/1 -> icub2deg/1
  icub2deg1/1 -> ms to s/1
  Cast To Single/1 -> icub2deg1/1
  icub2deg/1 -> position/1  "position"
  velocity raw/1 -> Cast To Single/1
  position raw/1 -> Cast To Single1/1
  ms to s/1 -> velocity/1  "velocity"

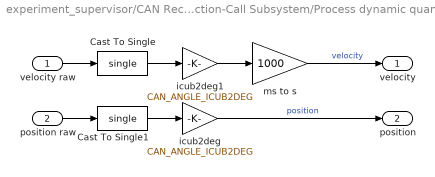
== system experiment_supervisor/CAN Receiver/Function-Call Subsystem/Process dynamic quantities1 ==
  velocity raw : Inport
  position raw : Inport  Port=2
  Cast To Single : DataTypeConversion  OutDataTypeStr=single  SaturateOnIntegerOverflow=off  RndMeth=Floor
  Cast To Single1 : DataTypeConversion  OutDataTypeStr=single  SaturateOnIntegerOverflow=off  RndMeth=Floor
  icub2deg : Gain  Gain=CAN_ANGLE_ICUB2DEG
  icub2deg1 : Gain  Gain=CAN_ANGLE_ICUB2DEG
  ms to s : Gain  Gain=1000
  velocity : Outport
  position : Outport  Port=2
  wires:
  Cast To Single1/1 -> icub2deg/1
  icub2deg1/1 -> ms to s/1
  Cast To Single/1 -> icub2deg1/1
  icub2deg/1 -> position/1  "position"
  velocity raw/1 -> Cast To Single/1
  position raw/1 -> Cast To Single1/1
  ms to s/1 -> velocity/1  "velocity"

== system experiment_supervisor/CAN Receiver/Function-Call Subsystem/convert Vq ==
  vq raw : Inport
  Data Type Conversion : DataTypeConversion  OutDataTypeStr=int16  SaturateOnIntegerOverflow=off  RndMeth=Floor
  Data Type Conversion1 : DataTypeConversion  OutDataTypeStr=single  SaturateOnIntegerOverflow=off  RndMeth=Floor
  Gain : Gain  Gain=1/32
  Gain1 : Gain  Gain=1/10
  vq : Outport
  wires:
  vq raw/1 -> Data Type Conversion/1
  Gain/1 -> Data Type Conversion1/1
  Data Type Conversion/1 -> Gain/1  "vq"
  Data Type Conversion1/1 -> Gain1/1
  Gain1/1 -> vq/1

== system experiment_supervisor/CAN Receiver/Function-Call Subsystem/convert Vq1 ==
  vq raw : Inport
  Data Type Conversion : DataTypeConversion  OutDataTypeStr=int16  SaturateOnIntegerOverflow=off  RndMeth=Floor
  Data Type Conversion1 : DataTypeConversion  OutDataTypeStr=single  SaturateOnIntegerOverflow=off  RndMeth=Floor
  Gain : Gain  Gain=1/32
  Gain1 : Gain  Gain=1/10
  vq : Outport
  wires:
  vq raw/1 -> Data Type Conversion/1
  Gain/1 -> Data Type Conversion1/1
  Data Type Conversion/1 -> Gain/1  "vq"
  Data Type Conversion1/1 -> Gain1/1
  Gain1/1 -> vq/1

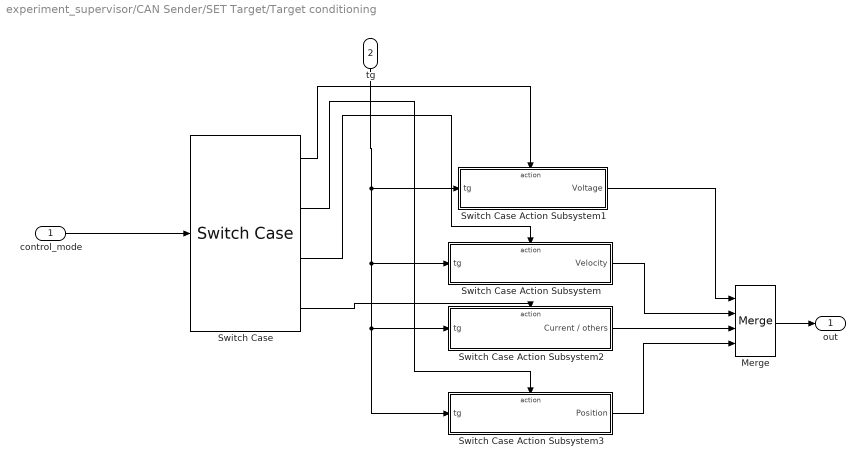
== system experiment_supervisor/CAN Sender/SET Target/Target conditioning ==
  control_mode : Inport
  tg : Inport  Port=2
  Merge : Merge  Inputs=4
  Switch Case : SwitchCase  CaseConditions={MCControlModes.OpenLoop,MCControlModes.Position ,MCControlModes.SpeedVoltage}
  Switch Case Action Subsystem : Subsystem  TreatAsAtomicUnit=on
  Switch Case Action Subsystem1 : Subsystem  TreatAsAtomicUnit=on
  Switch Case Action Subsystem2 : Subsystem  TreatAsAtomicUnit=on
  Switch Case Action Subsystem3 : Subsystem  TreatAsAtomicUnit=on
  out : Outport
  wires:
  tg/1 -> Switch Case Action Subsystem3/1(tg), Switch Case Action Subsystem2/1(tg), Switch Case Action Subsystem/1(tg), Switch Case Action Subsystem1/1(tg)
  Switch Case/1 -> Switch Case Action Subsystem1/Action
  Switch Case/4 -> Switch Case Action Subsystem2/Action
  Merge/1 -> out/1
  control_mode/1 -> Switch Case/1
  Switch Case Action Subsystem1/1(Voltage) -> Merge/1
  Switch Case Action Subsystem/1(Velocity) -> Merge/2
  Switch Case Action Subsystem2/1(Current / others) -> Merge/3
  Switch Case/2 -> Switch Case Action Subsystem3/Action
  Switch Case/3 -> Switch Case Action Subsystem/Action
  Switch Case Action Subsystem3/1(Position) -> Merge/4

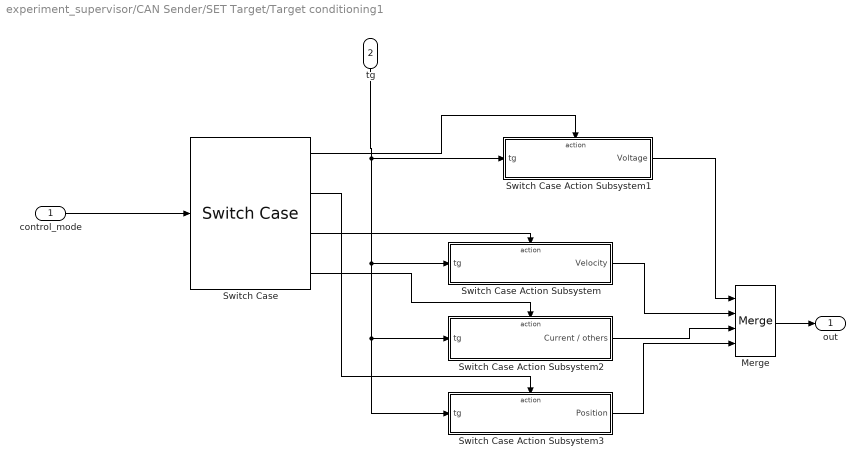
== system experiment_supervisor/CAN Sender/SET Target/Target conditioning1 ==
  control_mode : Inport
  tg : Inport  Port=2
  Merge : Merge  Inputs=4
  Switch Case : SwitchCase  CaseConditions={MCControlModes.OpenLoop,MCControlModes.Position ,MCControlModes.SpeedVoltage}
  Switch Case Action Subsystem : Subsystem  TreatAsAtomicUnit=on
  Switch Case Action Subsystem1 : Subsystem  TreatAsAtomicUnit=on
  Switch Case Action Subsystem2 : Subsystem  TreatAsAtomicUnit=on
  Switch Case Action Subsystem3 : Subsystem  TreatAsAtomicUnit=on
  out : Outport
  wires:
  Switch Case/1 -> Switch Case Action Subsystem1/Action
  Switch Case Action Subsystem3/1(Position) -> Merge/4
  Switch Case/3 -> Switch Case Action Subsystem/Action
  Switch Case/2 -> Switch Case Action Subsystem3/Action
  tg/1 -> Switch Case Action Subsystem3/1(tg), Switch Case Action Subsystem2/1(tg), Switch Case Action Subsystem/1(tg), Switch Case Action Subsystem1/1(tg)
  Switch Case Action Subsystem2/1(Current / others) -> Merge/3
  Merge/1 -> out/1
  Switch Case Action Subsystem/1(Velocity) -> Merge/2
  control_mode/1 -> Switch Case/1
  Switch Case/4 -> Switch Case Action Subsystem2/Action
  Switch Case Action Subsystem1/1(Voltage) -> Merge/1

== system experiment_supervisor/CAN Sender/SET Target POS /Target conditioning ==
  tg : Inport
  Zero : Constant  OutDataTypeStr=uint16
  ID : Outport
  Position : Outport  Port=2
  wires:
  Zero/1 -> ID/1
  tg/1 -> Position/1

== system experiment_supervisor/CAN Sender/Set Parameter/If Action Subsystem ==
  v : Inport
  ID : Inport  Port=2
  Action Port : ActionPort  ActionPortLabel=case [ elect_vmax ]:
  CAN Pack : canmsglib/CAN Pack  MsgList=(none)  MsgName=Set Value  MsgIDType=Standard (11-bit identifier)  MsgIdentifier=board_ID  CANIDInput=on  MsgLength=8  Remote=off  ApplyMinMax=off  BusOutput=on  SignalInfo={ 'OPC', '0', '8', 'LE', 'unsigned', 'Standard', '0', '1', '0', '-Inf', 'Inf'; 'value', '16', '32', 'LE', 'single', 'Standard', '0', '1', '0', '-Inf', 'Inf'; 'elec_vmax', '8', '8', 'LE', 'unsigned', 'Standard', '0', '1', '0', '-Inf', 'Inf' }
      settings: LibrarySourceBlock=stmutilitieslib/CAN Pack  DataFormat=manually specified signals
  Cast : DataTypeConversion  OutDataTypeStr=uint8  SaturateOnIntegerOverflow=off  RndMeth=Floor
  SET : Constant  Value=0x01  OutDataTypeStr=uint8
  elect_Vmax : Constant  Value=0x03  OutDataTypeStr=uint8
  m : Outport
  wires:
  v/1 -> Cast/1
  SET/1 -> CAN Pack/1
  ID/1 -> CAN Pack/4
  CAN Pack/1 -> m/1
  Cast/1 -> CAN Pack/2
  elect_Vmax/1 -> CAN Pack/3

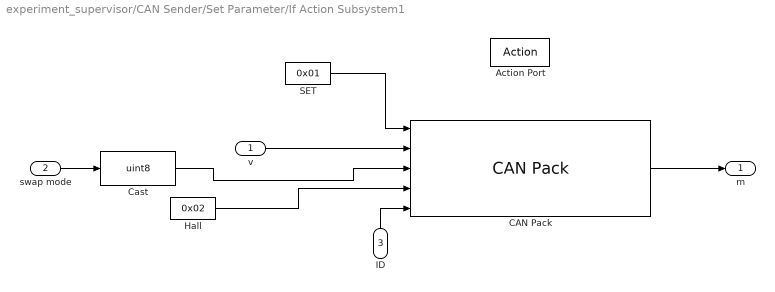
== system experiment_supervisor/CAN Sender/Set Parameter/If Action Subsystem1 ==
  v : Inport
  swap mode : Inport  Port=2
  ID : Inport  Port=3
  Action Port : ActionPort  ActionPortLabel=case [ hall ]:
  CAN Pack : canmsglib/CAN Pack  MsgList=(none)  MsgName=Set Value  MsgIDType=Standard (11-bit identifier)  MsgIdentifier=board_ID  CANIDInput=on  MsgLength=8  Remote=off  ApplyMinMax=off  BusOutput=on  SignalInfo={ 'OPC', '0', '8', 'LE', 'unsigned', 'Standard', '0', '1', '0', '-Inf', 'Inf'; 'offset', '16', '16', 'LE', 'unsigned', 'Standard', '0', '1', '0', '-Inf', 'Inf'; 'swap_mode', '32', '8', 'LE', 'unsigned', 'Standard', '0', '1', '0', '-Inf', 'Inf'; 'hall', '8', '8', 'LE', 'unsigned', 'Standard', '0', '1', '0', '-Inf', 'Inf' }
      settings: LibrarySourceBlock=stmutilitieslib/CAN Pack  DataFormat=manually specified signals
  Cast : DataTypeConversion  OutDataTypeStr=uint8  SaturateOnIntegerOverflow=off  RndMeth=Floor
  Hall : Constant  Value=0x02  OutDataTypeStr=uint8
  SET : Constant  Value=0x01  OutDataTypeStr=uint8
  m : Outport
  wires:
  CAN Pack/1 -> m/1
  SET/1 -> CAN Pack/1
  v/1 -> CAN Pack/2
  ID/1 -> CAN Pack/5
  swap mode/1 -> Cast/1
  Cast/1 -> CAN Pack/3
  Hall/1 -> CAN Pack/4

== system experiment_supervisor/CAN Sender/Set Parameter/If Action Subsystem2 ==
  v : Inport
  ID : Inport  Port=2
  Action Port : ActionPort  ActionPortLabel=case [ Kbemf ]:
  CAN Pack : canmsglib/CAN Pack  MsgList=(none)  MsgName=Set Value  MsgIDType=Standard (11-bit identifier)  MsgIdentifier=board_ID  CANIDInput=on  MsgLength=8  Remote=off  ApplyMinMax=off  BusOutput=on  SignalInfo={ 'OPC', '0', '8', 'LE', 'unsigned', 'Standard', '0', '1', '0', '-Inf', 'Inf'; 'value', '16', '32', 'LE', 'single', 'Standard', '0', '1', '0', '-Inf', 'Inf'; 'kbemf', '8', '8', 'LE', 'unsigned', 'Standard', '0', '1', '0', '-Inf', 'Inf' }
      settings: LibrarySourceBlock=stmutilitieslib/CAN Pack  DataFormat=manually specified signals
  Kbemf : Constant  Value=0x01  OutDataTypeStr=uint8
  SET : Constant  Value=0x01  OutDataTypeStr=uint8
  m : Outport
  wires:
  CAN Pack/1 -> m/1
  SET/1 -> CAN Pack/1
  v/1 -> CAN Pack/2
  ID/1 -> CAN Pack/4
  Kbemf/1 -> CAN Pack/3

== system experiment_supervisor/CAN Sender/SET Target/Target conditioning/Switch Case Action Subsystem ==
  tg : Inport
  Action Port : ActionPort  ActionPortLabel=case [ SpeedVoltage ]:
  Data Type Conversion2 : DataTypeConversion  OutDataTypeStr=int16  SaturateOnIntegerOverflow=off  RndMeth=Floor
  Gain : Gain  Gain=1/1000
  Product : Product
  deg2icub : Constant  Value=CAN_ANGLE_DEG2ICUB  OutDataTypeStr=single
  Velocity : Outport
  wires:
  tg/1 -> Product/2
  Gain/1 -> Product/1
  deg2icub/1 -> Gain/1
  Product/1 -> Data Type Conversion2/1
  Data Type Conversion2/1 -> Velocity/1

== system experiment_supervisor/CAN Sender/SET Target/Target conditioning/Switch Case Action Subsystem1 ==
  tg : Inport
  Action Port : ActionPort  ActionPortLabel=case [ OpenLoop ]:
  Data Type Conversion : DataTypeConversion  OutDataTypeStr=int16  SaturateOnIntegerOverflow=off  RndMeth=Floor
  Gain : Gain  Gain=32
  Gain1 : Gain  Gain=10
  Voltage : Outport
  wires:
  Gain1/1 -> Gain/1
  tg/1 -> Gain1/1
  Data Type Conversion/1 -> Voltage/1
  Gain/1 -> Data Type Conversion/1

== system experiment_supervisor/CAN Sender/SET Target/Target conditioning/Switch Case Action Subsystem2 ==
  tg : Inport
  Action Port : ActionPort  ActionPortLabel=default:
  Data Type Conversion3 : DataTypeConversion  OutDataTypeStr=int16  SaturateOnIntegerOverflow=off  RndMeth=Floor
  Current / others : Outport
  wires:
  tg/1 -> Data Type Conversion3/1
  Data Type Conversion3/1 -> Current / others/1

== system experiment_supervisor/CAN Sender/SET Target/Target conditioning/Switch Case Action Subsystem3 ==
  tg : Inport
  Action Port : ActionPort  ActionPortLabel=case [ Position ]:
  Data Type Conversion2 : DataTypeConversion  OutDataTypeStr=int16  SaturateOnIntegerOverflow=off  RndMeth=Floor
  Product : Product
  deg2icub : Constant  Value=CAN_ANGLE_DEG2ICUB  OutDataTypeStr=single
  Position : Outport
  wires:
  deg2icub/1 -> Product/1
  Product/1 -> Data Type Conversion2/1
  Data Type Conversion2/1 -> Position/1
  tg/1 -> Product/2

== system experiment_supervisor/CAN Sender/SET Target/Target conditioning1/Switch Case Action Subsystem ==
  tg : Inport
  Action Port : ActionPort  ActionPortLabel=case [ SpeedVoltage ]:
  Data Type Conversion2 : DataTypeConversion  OutDataTypeStr=int16  SaturateOnIntegerOverflow=off  RndMeth=Floor
  Gain : Gain  Gain=1/1000
  Product : Product
  deg2icub : Constant  Value=CAN_ANGLE_DEG2ICUB  OutDataTypeStr=single
  Velocity : Outport
  wires:
  tg/1 -> Product/2
  Gain/1 -> Product/1
  deg2icub/1 -> Gain/1
  Product/1 -> Data Type Conversion2/1
  Data Type Conversion2/1 -> Velocity/1

== system experiment_supervisor/CAN Sender/SET Target/Target conditioning1/Switch Case Action Subsystem1 ==
  tg : Inport
  Action Port : ActionPort  ActionPortLabel=case [ OpenLoop ]:
  Data Type Conversion : DataTypeConversion  OutDataTypeStr=int16  SaturateOnIntegerOverflow=off  RndMeth=Floor
  Gain : Gain  Gain=32
  Gain1 : Gain  Gain=10
  Voltage : Outport
  wires:
  Gain1/1 -> Gain/1
  tg/1 -> Gain1/1
  Data Type Conversion/1 -> Voltage/1
  Gain/1 -> Data Type Conversion/1

== system experiment_supervisor/CAN Sender/SET Target/Target conditioning1/Switch Case Action Subsystem2 ==
  tg : Inport
  Action Port : ActionPort  ActionPortLabel=default:
  Data Type Conversion3 : DataTypeConversion  OutDataTypeStr=int16  SaturateOnIntegerOverflow=off  RndMeth=Floor
  Current / others : Outport
  wires:
  tg/1 -> Data Type Conversion3/1
  Data Type Conversion3/1 -> Current / others/1

== system experiment_supervisor/CAN Sender/SET Target/Target conditioning1/Switch Case Action Subsystem3 ==
  tg : Inport
  Action Port : ActionPort  ActionPortLabel=case [ Position ]:
  Data Type Conversion2 : DataTypeConversion  OutDataTypeStr=int16  SaturateOnIntegerOverflow=off  RndMeth=Floor
  Product : Product
  deg2icub : Constant  Value=CAN_ANGLE_DEG2ICUB  OutDataTypeStr=single
  Position : Outport
  wires:
  tg/1 -> Product/2
  deg2icub/1 -> Product/1
  Product/1 -> Data Type Conversion2/1
  Data Type Conversion2/1 -> Position/1

== matlab function experiment_supervisor/CAN Sender/SET Target POS /MATLAB Function ==
  data: u input; y output
function y = single2hex(u)
in = half(u);
c= typecast(in,'uint16');
y = c;

== matlab function experiment_supervisor/CAN Sender/SET Motor config/Unpack motor configuration ==
  data: flags output; resolution output; rotor_offset output int16; n_poles output; motor_cfg input; enc_tolerance output
 function [flags, resolution,rotor_offset, n_poles, enc_tolerance] = unpack_cfg(motor_cfg)

    flags = uint8(motor_cfg.has_quadrature_encoder); 
    flags = bitor(flags, bitshift(uint8(motor_cfg.has_hall_sens), 1));
    resolution = motor_cfg.rotor_encoder_resolution;
    rotor_offset = motor_cfg.rotor_index_offset;
    n_poles = motor_cfg.pole_pairs * 2;
    enc_tolerance = motor_cfg.encoder_tolerance;

end
